simulink model "DC_MotorEquation_Encoder"  (R2024b)
settings: Solver=VariableStepAuto  StartTime=0.0  StopTime=0.1  FixedStep=0.0001  RelTol=1e-3
values from neighbouring files (symbols this model uses):
  b = 0    [DC_MotorEquation_Encoder_Parameters.m]    (also in param.m = 0.000180072449898)
  J = 0.352e-4    (= 3.52e-05)    [DC_MotorEquation_Encoder_Parameters.m]    (also in param.m)
  Km = 0.11    [DC_MotorEquation_Encoder_Parameters.m]    (also in param.m)
  L = 4.1e-3    (= 0.0041)    [DC_MotorEquation_Encoder_Parameters.m]    (also in param.m)
  PulseNumber = 2048*4    (= 8192)    [BaseModelForControl_Parameters.m]    (also in DC_MotorEquation_Encoder_Parameters.m)
  R = 3.2    [DC_MotorEquation_Encoder_Parameters.m]    (also in param.m)
  RadiantsPerCount = 2*pi/(PulseNumber-1)    (= 0.00076708403213)    [BaseModelForControl_Parameters.m]    (also in DC_MotorEquation_Encoder_Parameters.m)
  RadToRpm = 60/(2*pi)    (= 9.54929658551)    [BaseModelForControl_Parameters.m]    (also in DC_MotorEquation_Encoder_Parameters.m; param.m)
  TSample = PWM_Period    (= 0.0001)    [BaseModelForControl_Parameters.m]    (also in DC_MotorEquation_Encoder_Parameters.m)
settings Model: Creator=Davide  LastModifiedBy=student
settings DataIOCC: ReturnWorkspaceOutputs=off
settings OptimizationCC: ReuseModelBlockBuffer=off
settings RTWCC: GPUComputeCapability=3.5

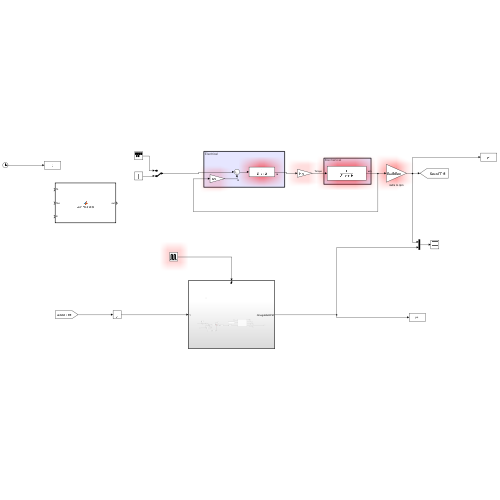
[thumbnail: Simulink's stored preview of the top-level diagram]
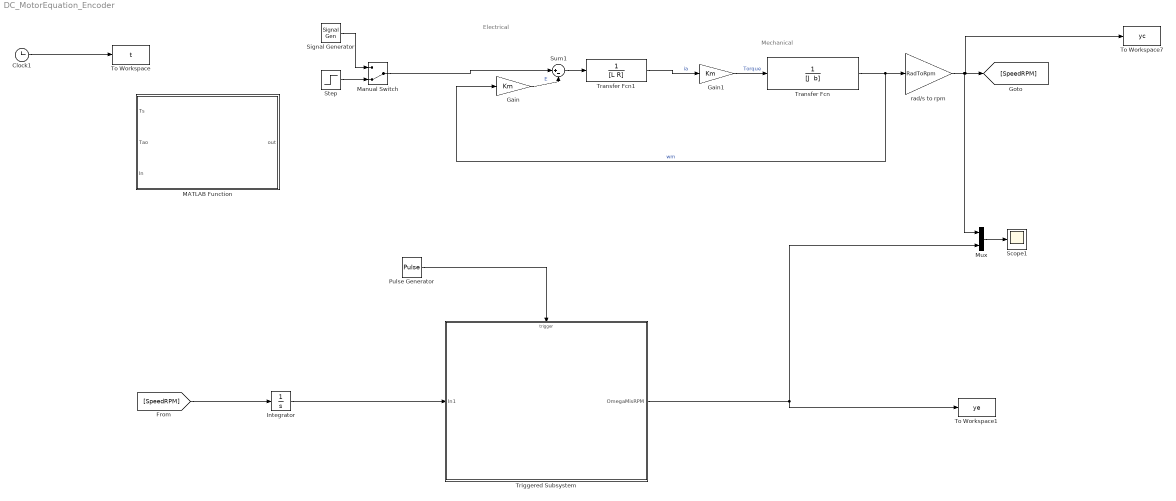
== system DC_MotorEquation_Encoder ==
  note: Electrical
  note: Mechanical
  Clock1 : Clock
  Gain : Gain  Gain=Km
  Gain1 : Gain  Gain=Km
  Integrator : Integrator
  MATLAB Function : MATLAB Function  TreatAsAtomicUnit=on
  Manual Switch : ManualSwitch  CurrentSetting=0
  Mux : Mux  Inputs=2
  Pulse Generator : DiscretePulseGenerator  PulseType=Time based  Period=TSample  PulseWidth=50
  Scope1 : Scope
  Signal Generator : SignalGenerator  WaveForm=square  Frequency=0.05
  Step : Step  Time=0  After=12  SampleTime=0
  Sum1 : Sum  Inputs=|+-
  To Workspace : ToWorkspace  VariableName=t  SampleTime=-1
  To Workspace1 : ToWorkspace  VariableName=ye  SampleTime=-1
  To Workspace7 : ToWorkspace  VariableName=yc  SampleTime=-1
  Transfer Fcn : TransferFcn  Denominator="[J  b]"
  Transfer Fcn1 : TransferFcn  Denominator=[L R]
  Triggered Subsystem : Subsystem  TreatAsAtomicUnit=on
  rad/s to rpm : Gain  Gain=RadToRpm  SaturateOnIntegerOverflow=on  OutDataTypeStr=Inherit: Same as input  ParamDataTypeStr=Inherit: Same as input
  wires:
  Signal Generator/1 -> Manual Switch/1
  Gain1/1 -> Transfer Fcn/1  "Torque"
  Transfer Fcn/1 -> Gain/1, rad/s to rpm/1  "wm"
  Transfer Fcn1/1 -> Gain1/1  "ia"
  Sum1/1 -> Transfer Fcn1/1
  Gain/1 -> Sum1/2  "E"
  Pulse Generator/1 -> Triggered Subsystem/Trigger
  Integrator/1 -> Triggered Subsystem/1(In1)
  [SpeedRPM] -> Integrator/1
  Step/1 -> Manual Switch/2
  Manual Switch/1 -> Sum1/1
  rad/s to rpm/1 -> To Workspace7/1, [SpeedRPM], Mux/1
  Triggered Subsystem/1(OmegaMisRPM) -> To Workspace1/1, Mux/2
  Mux/1 -> Scope1/1
  Clock1/1 -> To Workspace/1

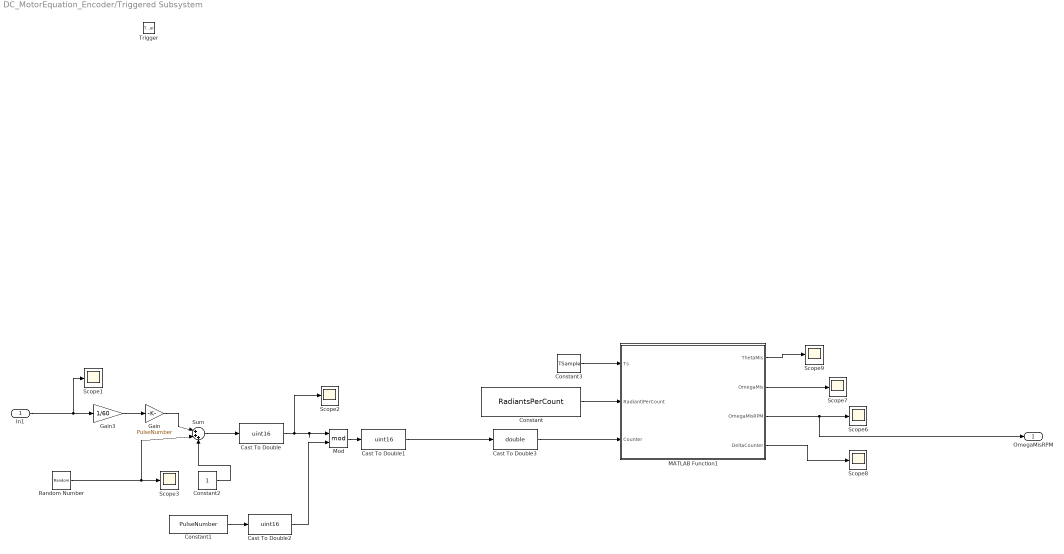
== system DC_MotorEquation_Encoder/Triggered Subsystem ==
  In1 : Inport
  Trigger : TriggerPort  VariantControl=(inherit)
  Cast To Double : DataTypeConversion  OutDataTypeStr=uint16  SaturateOnIntegerOverflow=off  RndMeth=Floor
  Cast To Double1 : DataTypeConversion  OutDataTypeStr=uint16  SaturateOnIntegerOverflow=off  RndMeth=Floor
  Cast To Double2 : DataTypeConversion  OutDataTypeStr=uint16  SaturateOnIntegerOverflow=off  RndMeth=Floor
  Cast To Double3 : DataTypeConversion  OutDataTypeStr=double  SaturateOnIntegerOverflow=off  RndMeth=Floor
  Constant : Constant  Value=RadiantsPerCount
  Constant1 : Constant  Value=PulseNumber
  Constant2 : Constant
  Constant3 : Constant  Value=TSample
  Gain : Gain  Gain=PulseNumber
  Gain3 : Gain  Gain=1/60
  MATLAB Function1 : MATLAB Function  TreatAsAtomicUnit=on
  Mod : Math  Operator=mod
  Random Number : RandomNumber  Variance=0.3
  Scope{1..3,6..9} (7 alike) : Scope
  Sum : Sum  Inputs=|+++
  OmegaMisRPM : Outport
  wires:
  Cast To Double2/1 -> Mod/2
  Cast To Double/1 -> Scope2/1, Mod/1
  Constant1/1 -> Cast To Double2/1
  Mod/1 -> Cast To Double1/1
  Cast To Double1/1 -> Cast To Double3/1
  Gain/1 -> Sum/1
  Constant/1 -> MATLAB Function1/2(RadiantiPerCount)
  Constant3/1 -> MATLAB Function1/1(Ts)
  MATLAB Function1/3(OmegaMisRPM) -> OmegaMisRPM/1, Scope6/1
  Cast To Double3/1 -> MATLAB Function1/3(Counter)
  MATLAB Function1/1(ThetaMis) -> Scope9/1
  MATLAB Function1/2(OmegaMis) -> Scope7/1
  MATLAB Function1/4(DeltaCounter) -> Scope8/1
  Gain3/1 -> Gain/1
  In1/1 -> Scope1/1, Gain3/1
  Sum/1 -> Cast To Double/1
  Random Number/1 -> Scope3/1, Sum/2
  Constant2/1 -> Sum/3

== matlab function DC_MotorEquation_Encoder/MATLAB Function ==
  data: Ts input; out output; Tao input; In input
function out  = LowPassFilter (Ts, Tao, In)

persistent OutPrecedente
if isempty(OutPrecedente)
    OutPrecedente = 0;
end
    %Filtro passa basso discretizzato con
    %il metodo delle differenze all'indietro

    a=Ts/(Ts+Tao);
    b=Tao/(Ts+Tao);

    out=a*In+OutPrecedente*b;
    OutPrecedente = out;

end

== matlab function DC_MotorEquation_Encoder/Triggered Subsystem/MATLAB Function1 ==
  data: Ts input; ThetaMis output; RadiantiPerCount input; Counter input; OmegaMis output; OmegaMisRPM output; DeltaCounter output
function [ThetaMis, OmegaMis, OmegaMisRPM, DeltaCounter] = CounterToThetaOmega(Ts, RadiantiPerCount, Counter)

% Inizializzazione dei valori iniziali 
persistent CounterPrec  
if isempty( CounterPrec )
    CounterPrec = 0;
end 

    DeltaCounter=Counter-CounterPrec;
    
    if (DeltaCounter>double(0x1000))
        DeltaCounter=DeltaCounter-double(0x2000);
    end
    
    if (DeltaCounter<-double(0x1000))
        DeltaCounter=DeltaCounter+double(0x2000);
    end
        
    % conversione conteggio in radianti
    ThetaMis = Counter * RadiantiPerCount;
    
    DeltaThetaMis = DeltaCounter*RadiantiPerCount;
   
    OmegaMis = DeltaThetaMis/Ts;
    OmegaMisRPM=OmegaMis*60/(2*pi);
 
    CounterPrec= Counter;
end
